simulink model "vita_sys_06"  (R2025b)
settings: Solver=VariableStepAuto  StartTime=0.0  StopTime=10.0  RelTol=1e-3
libraries: autolibshared x1, vehdynlibdriver x1, drivingscenarioandsensors x1
settings Model: Creator=ADMIIN  LastModifiedBy=ADMIIN

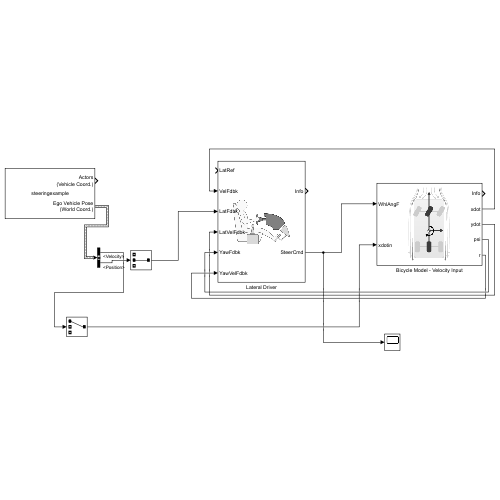
[thumbnail: Simulink's stored preview of the top-level diagram]
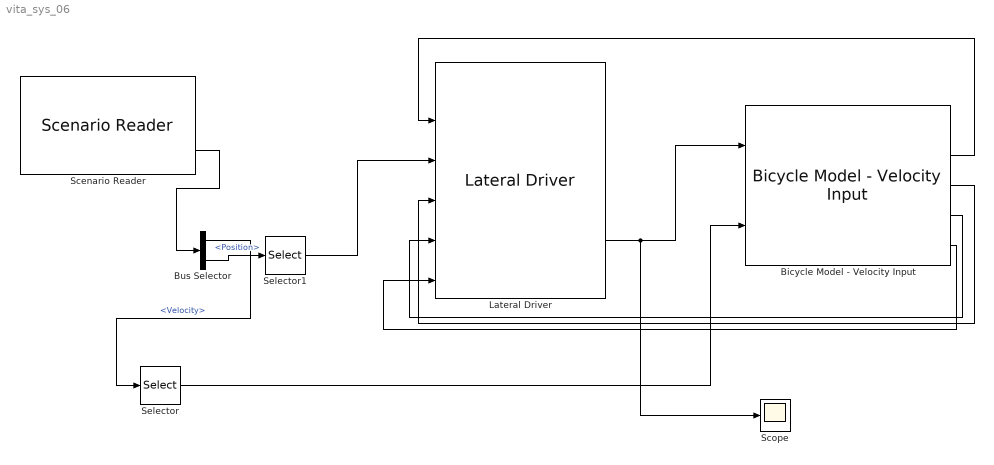
== system vita_sys_06 ==
  Bicycle Model - Velocity Input : autolibshared/Bicycle Model - Velocity Input  trackMode=Single (bicycle)  inputMode=External longitudinal velocity  frontSteerMode=on  rearSteerMode=off  windMode=off  muMode=off  extFMode=off  extMMode=off  aMode=3  NF=2  NR=2  m=2000  a=1.4  b=1.6  h=0.35  X_o=0  xdot_o=0  CalphaMode=off  sigmaMode=on  w=[1.4,1.4]  Cy_f=12e3  Cy_r=11e3  sigma_f=.1  sigma_r=.1  alpha_f_brk=[-.1 .1]  Cy_f_data=[-9e3 9e3]  alpha_r_brk=[-.1 .1]  Cy_r_data=[-9e3 9e3]  Y_o=0  ydot_o=0  Izz=4000  psi_o=0  r_o=0  Af=2  Cd=.3  Cl=.1  Cpm=.1  beta_w=[0 0.01:0.01:0.3]  Cs=[0 0.01:0.01:0.3]  Cym=[0 1e-6:0.01:0.3]  Pabs=101325  Tair=273  g=9.81  mu=1  xdot_tol=.01  Fznom=5000  Fxtire_sat=1e6  Fytire_sat=1e6  longOff=0  latOff=0  vertOff=0
      settings: LibrarySourceBlock=drivingscenarioandsensors/Bicycle Model - Velocity Input
  Bus Selector : BusSelector  OutputSignals=Velocity,Position
  Lateral Driver : vehdynlibdriver/Lateral Driver  extSteerOvr=off  extSteerHld=off  extSteerZero=off  steerOut=off  cntrlTypeLat=Predictive  coordMode=SAE J670 (Z-down)  angUnits=rad  tau=0.1  L=3  vecPose=off  dynamMode=off  PositionGainF=2.5  PositionGainR=2.5  YawRateGain=.2  DelayGain=.2  a=1.41  b=1.41  m=2016  Cy_f=25266  Cy_r=70933  I=4013  Ksteer=18  theta=45*pi/180  aMode=2
  Scenario Reader : drivingscenarioandsensors/Scenario Reader  ScenarioSource=From file  ScenarioFileName=C:\Users\ADMIIN\OneDrive\Documents\MATLAB\Examples\R2025b\autonomous_control\AdaptiveCruiseControlWithSensorFusionExample\steeringexample.mat  ScenarioVariableName=scenario  OutputCoordinateSystem=Vehicle coordinates  EgoVehicleSource=Scenario  EgoVehicleActorID=1  OrientVehiclesOnRoad=off  OutputEgoVehiclePose=on  OutputEgoVehicleState=off  SampleTime=0.1  LaneBoundaryOutput=None  LaneBoundaryDistance=0:0.5:9.5  LaneBoundaryLocation=Center of lane markings  BusNameSource=Auto  BusName=BusActors  BusNumActorsSource=Scenario  BusNumActors=100  BusName2Source=Auto  BusName2=BusLaneBoundaries  BusNumLaneBoundariesSource=Scenario  BusNumLaneBoundaries=10  BusName3Source=Auto  BusName3=BusEgoActor  BusName4Source=Auto  BusName4=BusEgoState  ShowCoordinateLabels=on  SimulateUsing=Interpreted execution
  Scope : Scope
      settings: ActiveDisplayYMinimum=-1.2138159331775131  ActiveDisplayYMaximum=0.9243433985976186
  Selector : Selector  InputPortWidth=3  IndexOptions=Index vector (dialog)  Indices=[1]  OutputSizes=1
  Selector1 : Selector  InputPortWidth=3  IndexOptions=Index vector (dialog)  Indices=[2]  OutputSizes=1
  wires:
  Lateral Driver/2 -> Scope/1, Bicycle Model - Velocity Input/1
  Scenario Reader/2 -> Bus Selector/1
  Bus Selector/1 -> Selector/1  "<Velocity>"
  Bicycle Model - Velocity Input/2 -> Lateral Driver/2
  Bicycle Model - Velocity Input/3 -> Lateral Driver/4
  Bicycle Model - Velocity Input/4 -> Lateral Driver/5
  Bicycle Model - Velocity Input/5 -> Lateral Driver/6
  Selector/1 -> Bicycle Model - Velocity Input/2
  Bus Selector/2 -> Selector1/1  "<Position>"
  Selector1/1 -> Lateral Driver/3
